simulink model "OpenLoop"  (R2024b)
settings: Solver=VariableStepAuto  StartTime=0.0  StopTime=10.0  RelTol=1e-3
settings Model: Creator=RC 21.9.22  LastModifiedBy=RC 21.9.22

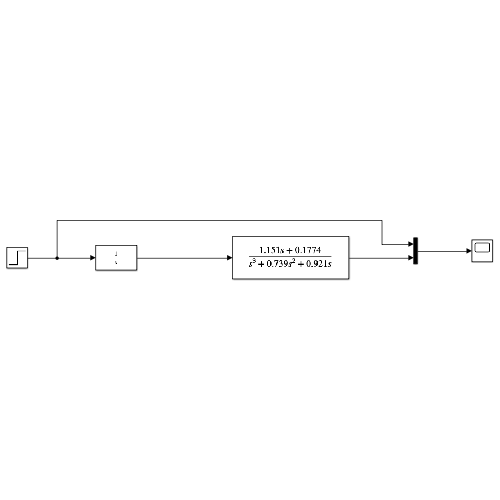
[thumbnail: Simulink's stored preview of the top-level diagram]
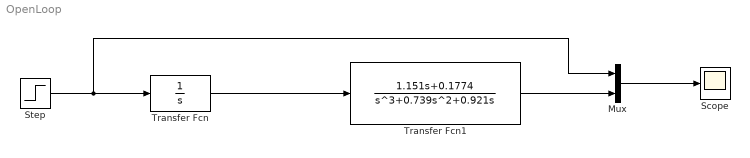
== system OpenLoop ==
  Mux : Mux  Inputs=2
  Scope : Scope
  Step : Step  Time=0.2  After=0.2  SampleTime=0
  Transfer Fcn : TransferFcn  Denominator=[1 0]
  Transfer Fcn1 : TransferFcn  Numerator=[1.151 0.1774]  Denominator=[1 0.739 0.921 0]
  wires:
  Transfer Fcn/1 -> Transfer Fcn1/1
  Step/1 -> Mux/1, Transfer Fcn/1
  Transfer Fcn1/1 -> Mux/2
  Mux/1 -> Scope/1
